simulink model "HPIPM_Interface"  (R2024a)
settings: Solver=FixedStepDiscrete  StartTime=0.0  StopTime=.2  FixedStep=.2  RelTol=1e-3
settings Model: Creator=zz  LastModifiedBy=zz

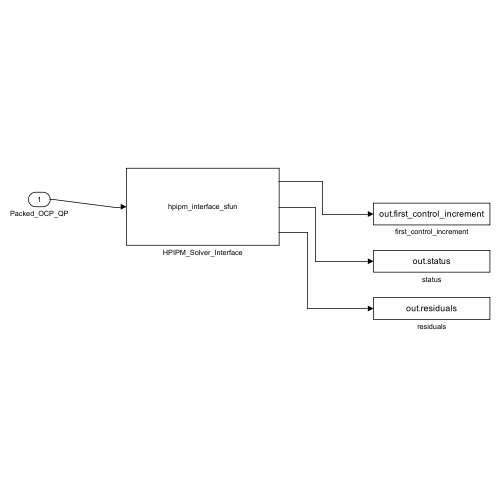
[thumbnail: Simulink's stored preview of the top-level diagram]
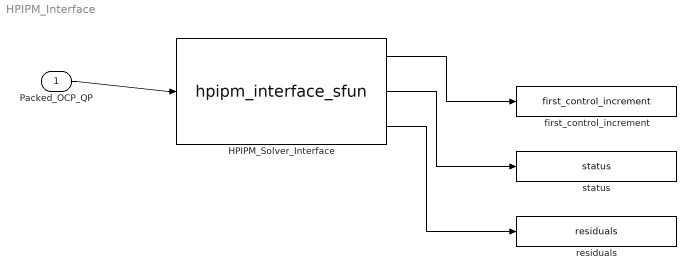
== system HPIPM_Interface ==
  Packed_OCP_QP : Inport  PortDimensions=9174
  HPIPM_Solver_Interface : M-S-Function  FunctionName=hpipm_interface_sfun
  first_control_increment : ToWorkspace  VariableName=first_control_increment  SaveFormat=Timeseries
  residuals : ToWorkspace  VariableName=residuals  SaveFormat=Timeseries
  status : ToWorkspace  VariableName=status  SaveFormat=Timeseries
  wires:
  Packed_OCP_QP/1 -> HPIPM_Solver_Interface/1
  HPIPM_Solver_Interface/1 -> first_control_increment/1
  HPIPM_Solver_Interface/2 -> status/1
  HPIPM_Solver_Interface/3 -> residuals/1
